simulink model "model_analysis_02"  (R2026b)
settings: Solver=VariableStepAuto  StopTime=30e-3
InitFcn:
  | parameters_current_control;
values from neighbouring files (symbols this model uses):
  Ki = Kp/Ti    (= 18750)    [parameters_current_control.m]    (also in sim_analysis_02_PI_controller.m = Kp/Ti; sim_analysis_02_P_controller.m = 0)
  Kp = Kp_norm*R    (= 75)    [parameters_current_control.m]    (also in sim_analysis_02_PI_controller.m = R*Kp_norm(k); sim_analysis_02_P_controller.m = R*Kp_norm(k))
  L = 6e-3    (= 0.006)    [parameters_current_control.m]
  R = 1.5    [parameters_current_control.m]
  Ts = 50e-6    (= 5e-05)    [parameters_current_control.m]
libraries: slpidlib x1
settings Model: Creator=ZAID  LastModifiedBy=ZAID

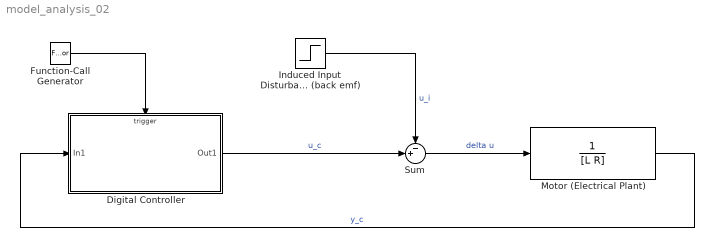
== system model_analysis_02 ==
  Digital Controller : Subsystem  TreatAsAtomicUnit=on
  Function-Call Generator : FunctionCallGenerator  SampleTime=Ts
  Induced Input Disturbance (back emf) : Step  Time=0  FinalValue=0.1  SampleTime=0
  Motor (Electrical Plant) : TransferFcn  Denominator=[L R]
  Sum : Sum  Inputs=-+|
  wires:
  Sum/1 -> Motor (Electrical Plant)/1  "delta u"
  Digital Controller/1(Out1) -> Sum/2  "u_c"
  Induced Input Disturbance (back emf)/1 -> Sum/1  "u_i"
  Motor (Electrical Plant)/1 -> Digital Controller/1(In1)  "y_c"
  Function-Call Generator/1 -> Digital Controller/Trigger

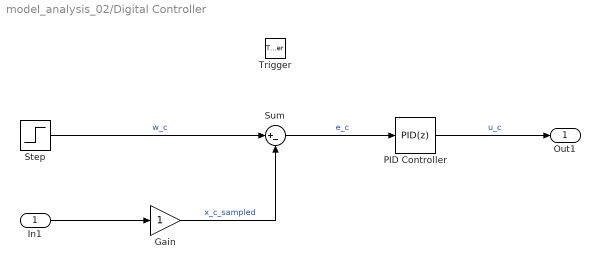
== system model_analysis_02/Digital Controller ==
  In1 : Inport
  Trigger : TriggerPort  TriggerType=function-call  VariantControl=(inherit)
  Gain : Gain
  PID Controller : slpidlib/PID Controller  Controller=PID  Form=Parallel  TimeDomain=Discrete-time  UseExternalTs=off  SampleTime=-1  IntegratorMethod=Forward Euler  FilterMethod=Forward Euler  ControllerParametersSource=internal  P=Kp  I=Ki  UseKiTs=off  D=0  UseExternalDerivativeSource=off  N=100  UseFilter=on  TunerSelectOption=Transfer Function Based (PID Tuner App)  InitialConditionSource=internal  InitialConditionForIntegrator=0  InitialConditionForFilter=0  DifferentiatorICPrevScaledInput=0  ExternalReset=none  TrackingMode=off  Kt=1  LimitOutput=off  SatLimitsSource=internal  UpperSaturationLimit=inf  LowerSaturationLimit=-inf  LinearizeAsGain=on  AntiWindupMode=none  Kb=1  LimitIntegrator=off  UpperIntegratorSaturationLimit=inf  LowerIntegratorSaturationLimit=-inf  POutMin=[]  POutMax=[]  IOutMin=[]  IOutMax=[]  DOutMin=[]  DOutMax=[]  NOutMin=[]  NOutMax=[]  SumOutMin=[]  SumOutMax=[]  SaturationOutMin=[]  SaturationOutMax=[]  PParamMin=[]  PParamMax=[]  IParamMin=[]  IParamMax=[]  DParamMin=[]  DParamMax=[]  NParamMin=[]  NParamMax=[]  KbParamMin=[]  KbParamMax=[]  KtParamMin=[]  KtParamMax=[]  KbOutMin=[]  KbOutMax=[]  KtOutMin=[]  KtOutMax=[]  IntegratorOutMin=[]  IntegratorOutMax=[]  FilterOutMin=[]  FilterOutMax=[]  SumI1OutMin=[]  SumI1OutMax=[]  SumI2OutMin=[]  SumI2OutMax=[]  SumI3OutMin=[]  SumI3OutMax=[]  SumI4OutMin=[]  SumI4OutMax=[]  SumDOutMin=[]  SumDOutMax=[]  DifferentiatorOutMin=[]  DifferentiatorOutMax=[]  FilterDiffOutCoefMin=[]  FilterDiffOutCoefMax=[]  ReciprocalOutMin=[]  ReciprocalOutMax=[]  SumDenOutMin=[]  SumDenOutMax=[]  SumNumOutMin=[]  SumNumOutMax=[]  DivideOutMin=[]  DivideOutMax=[]  UdiffTsProdOutMin=[]  UdiffTsProdOutMax=[]  NTsProdOutMin=[]  NTsProdOutMax=[]  UintegralTsProdOutMin=[]  UintegralTsProdOutMax=[]  UngainTsProdOutMin=[]  UngainTsProdOutMax=[]  ClampingZeroOutDataTypeStr=Inherit: Inherit via back propagation  ClampingZeroOutMin=[]  ClampingZeroOutMax=[]  FilterDenConstantOutDataTypeStr=Inherit: Inherit via back propagation  FilterDenConstantOutMin=[]  FilterDenConstantOutMax=[]  PCopyOutDataTypeStr=Inherit: Inherit via back propagation  PCopyOutMin=[]  PCopyOutMax=[]  NCopyOutDataTypeStr=Inherit: Inherit via back propagation  NCopyOutMin=[]  NCopyOutMax=[]  IntegratorContinuousStateAttributes=''  IntegratorStateMustResolveToSignalObject=off  IntegratorRTWStateStorageClass=Auto  FilterContinuousStateAttributes=''  FilterStateMustResolveToSignalObject=off  FilterRTWStateStorageClass=Auto  ParallelPVariant=InternalParameters  IdealPVariant=Disabled  IVariant=InternalParameters  DVariant=InternalParameters  IntegratorVariant=Discrete  SatVariant=Disabled  AWVariant=Passthrough  PCopyVariant=Disabled  TRVariant=Disabled  FdbkBlocksVariant=Forward  IdealPFdbkVariant=Disabled  SatFdbkVariant=Disabled  DerivativeFilterVariant=ForwardEulerFilter  NVariant=InternalParameters  NCopyVariant=Disabled  FilterICVariant=InternalICsFilter  IntegratorICVariant=InternalICs  ExternalResetVariant=Disabled  TRSumVariant=Passthrough  SumFdbkVariant=Disabled  SumVariant=Sum_PID  TsampFilterVariant=InternalTs  TsampNgainVariant=Passthrough  TsampIntegralVariant=Disabled_SignalSpec  ExternalSaturationOutDataTypeStr=Inherit: Same as second input  DerivativeSourceVariant=ErrorSignal  PreIntVariant=InternalPreInt
  Step : Step  Time=0
  Sum : Sum  Inputs=|+-
  Out1 : Outport
  wires:
  PID Controller/1 -> Out1/1  "u_c"
  Step/1 -> Sum/1  "w_c"
  Sum/1 -> PID Controller/1  "e_c"
  In1/1 -> Gain/1
  Gain/1 -> Sum/2  "x_c_sampled"
